simulink model "DC_Motor_FOPID_Auto"  (R2026b)
settings: Solver=VariableStepAuto  StopTime=10
values from neighbouring files (symbols this model uses):
  A_D = SD.A    [build_fopid_model.m]
  A_I = SI.A    [build_fopid_model.m]
  B = 0.2    [build_fopid_model.m]    (also in main_project.m)
  B_D = SD.B    [build_fopid_model.m]
  B_I = SI.B    [build_fopid_model.m]
  C_D = SD.C    [build_fopid_model.m]
  C_I = SI.C    [build_fopid_model.m]
  D_D = SD.D    [build_fopid_model.m]
  D_I = SI.D    [build_fopid_model.m]
  J = 0.02    [build_fopid_model.m]    (also in main_project.m)
  Kd = R.Kd_opt    [build_fopid_model.m]    (also in main_project.m = 0.5; optimize_fopid.m = x(3))
  Ke = 0.1    [build_fopid_model.m]    (also in main_project.m)
  Ki = R.Ki_opt    [build_fopid_model.m]    (also in main_project.m = 20; optimize_fopid.m = x(2))
  Kp = R.Kp_opt    [build_fopid_model.m]    (also in main_project.m = 10; optimize_fopid.m = x(1))
  Kt = 0.1    [build_fopid_model.m]    (also in main_project.m)
  La = 0.5    [build_fopid_model.m]    (also in main_project.m)
  Ra = 2    [build_fopid_model.m]    (also in main_project.m)
settings Model: Creator=Shobhit  LastModifiedBy=Shobhit

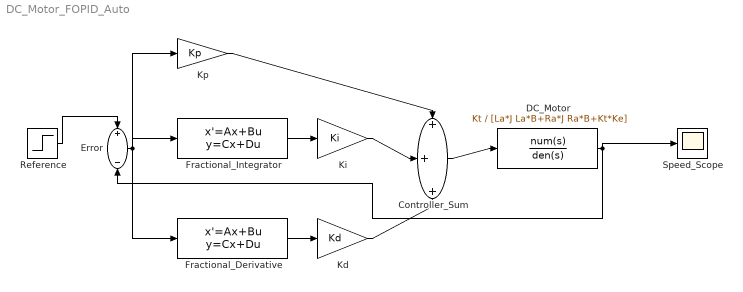
== system DC_Motor_FOPID_Auto ==
  Controller_Sum : Sum  Inputs=+++
  DC_Motor : TransferFcn  Numerator=Kt  Denominator=[La*J La*B+Ra*J Ra*B+Kt*Ke]
  Error : Sum  Inputs=+-
  Fractional_Derivative : StateSpace  A=A_D  B=B_D  C=C_D  D=D_D  InitialCondition=0
  Fractional_Integrator : StateSpace  A=A_I  B=B_I  C=C_I  D=D_I  InitialCondition=0
  Kd : Gain  Gain=Kd
  Ki : Gain  Gain=Ki
  Kp : Gain  Gain=Kp
  Reference : Step  Time=0  SampleTime=0
  Speed_Scope : Scope
  wires:
  Reference/1 -> Error/1
  Error/1 -> Kp/1, Fractional_Integrator/1, Fractional_Derivative/1
  Kp/1 -> Controller_Sum/1
  Fractional_Integrator/1 -> Ki/1
  Ki/1 -> Controller_Sum/2
  Fractional_Derivative/1 -> Kd/1
  Kd/1 -> Controller_Sum/3
  Controller_Sum/1 -> DC_Motor/1
  DC_Motor/1 -> Speed_Scope/1, Error/2
